simulink model "NGW_model"  (R2023b)
settings: Solver=ode4  StartTime=0  StopTime=0.5  FixedStep=1e-6  MaxStep=2e-4  RelTol=1e-7  AbsTol=1e-9
InitFcn:
  | NGW_init
values from neighbouring files (symbols this model uses):
  cL = 0    [NGW_init.m]    (also in NGW_test.m = 0.5)
  Flux = 0.01337    [NGW_init.m]
  i_ratio = p_m.i_ratio    [NGW_init.m]
  J_load = 4.53e-4    (= 0.000453)    [NGW_init.m]
  J_rotor = 1.0521e-4    (= 0.00010521)    [NGW_init.m]
  Kic = wc_i*1.05    (= 3298.67228627)    [NGW_init.m]
  Kis = Kps/Ti_s    [NGW_init.m]
  Kpc = wc_i*1.46e-3    (= 4.58672527424)    [NGW_init.m]
  Kps = wc_s*J_eq/Kt    [NGW_init.m]
  NtoW = 2*pi/60    (= 0.10471975512)    [NGW_init.m]
  P_n = 14    [NGW_init.m]
  TL_amp = 6    [NGW_init.m]
  TL_t0 = 0.2    [NGW_init.m]
  w_ref = 500    [NGW_init.m]
undefined symbols (not defined in the file or in its folder): NGW_params
libraries: slpidlib x6, spsDCVoltageSourceLib x2, spsUniversalBridgeLib x2, spsPermanentMagnetSynchronousMachineLib x2, spsSVPWMGenerator2LevelLib x2, sps_lib x1
settings Model: Creator=Administrator  LastModifiedBy=Administrator

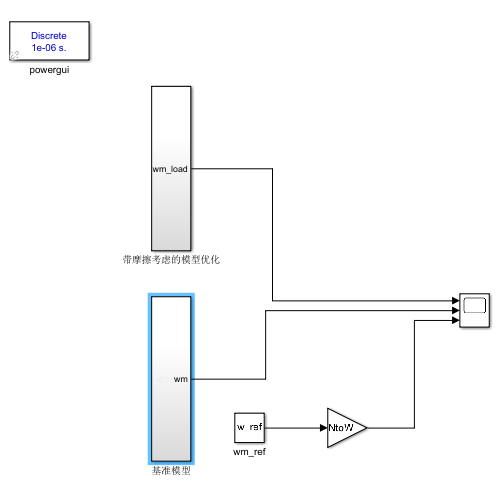
[thumbnail: Simulink's stored preview of the top-level diagram]
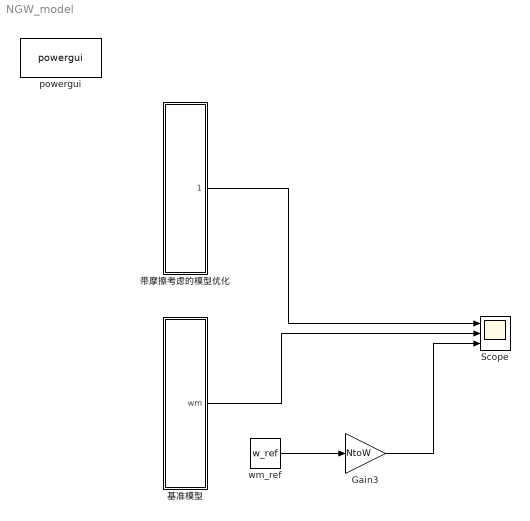
== system NGW_model ==
  Gain3 : Gain  Gain=NtoW
  Scope : Scope  NumInputPorts=3
  powergui : sps_lib/powergui  Priority=1  SimulationMode=Discrete  SampleTime=1e-6  frequency=60  Iterations=50  frequencyindice=0  Pbase=100e6  ErrMax=1e-4  UnitsV=kV  UnitsW=MW  buscounter=0  FunctionMessages=off  echomessages=off  EnableUseOfTLC=off  CurrentSourceSwitches=off  DisableSnubberDevices=off  DisableRonSwitches=off  DisableVfSwitches=off  DisplayEquations=off  AutomaticDiscreteSolvers=off  SolverType=Tustin/Backward Euler (TBE)  Interpol=off  ExternalGateDelay=off  methode=off  Ts=100  x0status=blocks  SPID=on  SwTol=0  HookPort=off  NonlinearTolerance=1e-4  nMaxIteration=100  ContinueOnMaxIteration=off  RestoreLinks=warning  ResistiveCurrentMeasurement=off  Frange=[0:2:500]  Ylog=off  Xlog=on  ShowGrid=off  save=off  variable=ZData  structure=0  ZoomFFT=off  StartTime=0.0  cycles=1  DisplayStyle=1  fundamental=60  FreqAxis=off  MaxFrequency=1000  frequencyindicesteady=1  RmsSteady=1  display=off
  wm_ref : Constant  Value=w_ref  SampleTime=-1
  基准模型 : Subsystem
  带摩擦考虑的模型优化 : Subsystem
  wires:
  带摩擦考虑的模型优化/1(wm_load) -> Scope/1
  基准模型/1(wm) -> Scope/2
  Gain3/1 -> Scope/3
  wm_ref/1 -> Gain3/1

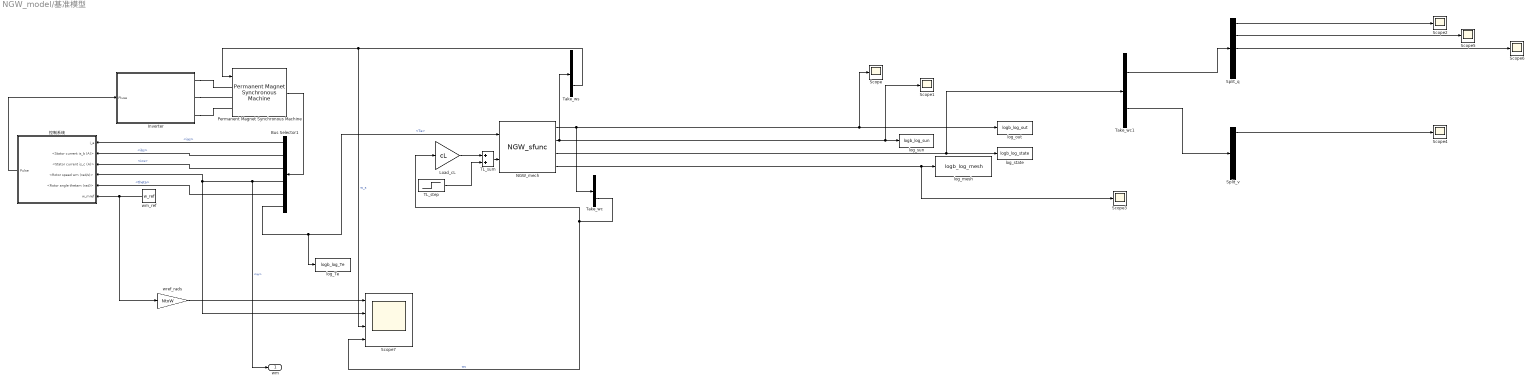
== system NGW_model/基准模型 ==
  Bus Selector1 : BusSelector  OutputSignals=ias,ibs,ics,w,theta,Te
  Inverter : Subsystem
  Load_cL : Gain  Gain=cL
  NGW_mech : M-S-Function  FunctionName=NGW_sfunc  Parameters=NGW_params(J_rotor, J_load)
  Permanent Magnet Synchronous Machine : spsPermanentMagnetSynchronousMachineLib/Permanent Magnet Synchronous Machine  NbPhases=3  FluxDistribution=Sinusoidal  RotorType=Round  MechanicalLoad=Speed w  PresetModel=No  ShowDetailedParameters=on  MeasurementBus=on  Resistance=1.05  Inductance=1.46e-3  dqInductances=[1.46e-3,1.46e-3]  La=0.000395  MachineConstant=Flux linkage established by magnets (V.s)  Flux=0.01337  VoltageCst=33.9507  TorqueCst=0.28077  Flat=120  Mechanical=[1.0521e-4 0 14 0]  PolePairs=14  InitialConditions=[0,0, 0,0]  InitialConditions5ph=[0 0 0 0 0 0]  RefAngle=Aligned with phase A axis (original Park)  IterativeDiscreteModel=Trapezoidal non iterative  TsBlock=-1  TsPowergui=0
  Scope{,1..6} (7 alike) : Scope
  Scope7 : Scope  NumInputPorts=4
  Split_q : Demux  Outputs=5
  Split_v : Demux  Outputs=5
  TL_step : Step  Time=TL_t0  After=TL_amp  SampleTime=0
  TL_sum : Sum
  Take_wc : Demux  Outputs=2
  Take_wc1 : Demux  Outputs=2
  Take_ws : Demux  Outputs=2
  log_Te : ToWorkspace  VariableName=logb_log_Te  SaveFormat=Timeseries  SampleTime=-1
  log_mesh : ToWorkspace  VariableName=logb_log_mesh  SaveFormat=Structure With Time  SampleTime=-1
  log_out : ToWorkspace  VariableName=logb_log_out  SaveFormat=Structure With Time  SampleTime=-1
  log_state : ToWorkspace  VariableName=logb_log_state  SaveFormat=Structure With Time  SampleTime=-1
  log_sun : ToWorkspace  VariableName=logb_log_sun  SaveFormat=Structure With Time  SampleTime=-1
  wm_ref : Constant  Value=w_ref  SampleTime=-1
  wref_rads : Gain  Gain=NtoW
  控制系统 : Subsystem
  wm : Outport
  wires:
  Split_v/1 -> Scope4/1
  Bus Selector1/5 -> 控制系统/5(<Rotor angle thetam (rad)>)  "<theta>"
  Split_q/2 -> Scope5/1
  Take_wc1/1 -> Split_q/1
  Bus Selector1/6 -> NGW_mech/1, log_Te/1  "<Te>"
  NGW_mech/1 -> log_out/1, Scope/1, Take_wc/1
  wm_ref/1 -> wref_rads/1, 控制系统/6(w_mref)
  Take_wc/2 -> Scope7/4, Load_cL/1  "wc"
  控制系统/1(Pulse) -> Inverter/1(Pluse)
  Take_wc1/2 -> Split_v/1
  Take_ws/2 -> Scope7/3, Permanent Magnet Synchronous Machine/1  "w_s"
  Split_q/1 -> Scope2/1
  Bus Selector1/1 -> 控制系统/1(i_a)  "<ias>"
  Split_q/3 -> Scope6/1
  NGW_mech/4 -> Scope3/1, log_mesh/1
  wref_rads/1 -> Scope7/1
  NGW_mech/2 -> Take_ws/1, Scope1/1, log_sun/1
  Bus Selector1/3 -> 控制系统/3(<Stator current is_c (A)>)  "<ics>"
  Bus Selector1/4 -> wm/1, Scope7/2, 控制系统/4(<Rotor speed wm (rad/s)>)  "<w>"
  NGW_mech/3 -> Take_wc1/1, log_state/1
  Permanent Magnet Synchronous Machine/1 -> Bus Selector1/1
  Bus Selector1/2 -> 控制系统/2(<Stator current is_b (A)>)  "<ibs>"
  Load_cL/1 -> TL_sum/1
  TL_step/1 -> TL_sum/2
  TL_sum/1 -> NGW_mech/2
  connections:
  Inverter/RConn2 -- Permanent Magnet Synchronous Machine/LConn2
  Inverter/RConn3 -- Permanent Magnet Synchronous Machine/LConn3
  Inverter/RConn1 -- Permanent Magnet Synchronous Machine/LConn1

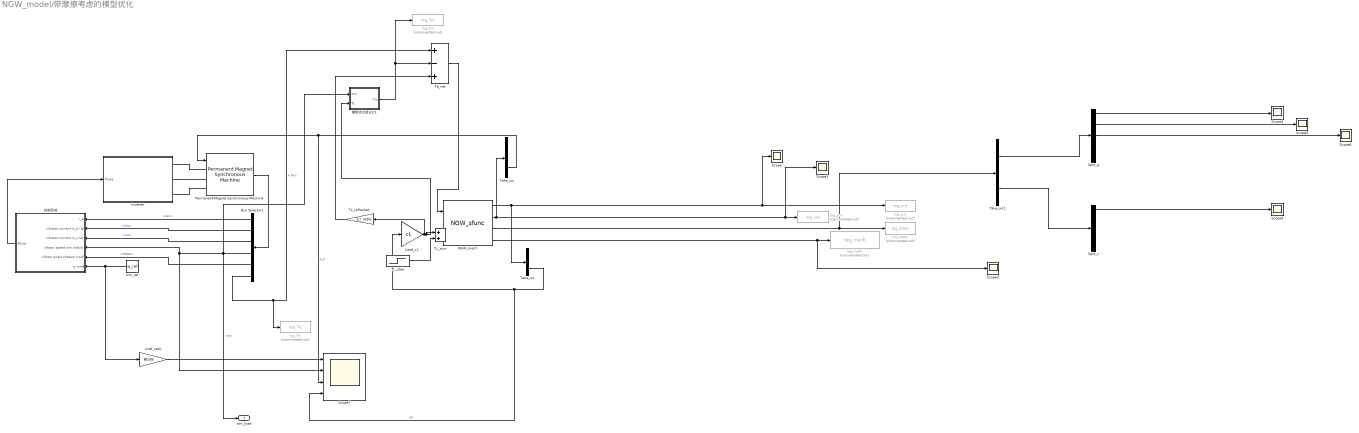
== system NGW_model/带摩擦考虑的模型优化 ==
  Bus Selector1 : BusSelector  OutputSignals=ias,ibs,ics,w,theta,Te
  Inverter : Subsystem
  Load_cL : Gain  Gain=cL
  NGW_mech : M-S-Function  FunctionName=NGW_sfunc  Parameters=NGW_params(J_rotor, J_load)
  Permanent Magnet Synchronous Machine : spsPermanentMagnetSynchronousMachineLib/Permanent Magnet Synchronous Machine  NbPhases=3  FluxDistribution=Sinusoidal  RotorType=Round  MechanicalLoad=Speed w  PresetModel=No  ShowDetailedParameters=on  MeasurementBus=on  Resistance=1.05  Inductance=1.46e-3  dqInductances=[1.46e-3,1.46e-3]  La=0.000395  MachineConstant=Flux linkage established by magnets (V.s)  Flux=0.01337  VoltageCst=33.9507  TorqueCst=0.28077  Flat=120  Mechanical=[1.0521e-4 0 14 0]  PolePairs=14  InitialConditions=[0,0, 0,0]  InitialConditions5ph=[0 0 0 0 0 0]  RefAngle=Aligned with phase A axis (original Park)  IterativeDiscreteModel=Trapezoidal non iterative  TsBlock=-1  TsPowergui=0
  Scope{,1..6} (7 alike) : Scope
  Scope7 : Scope  NumInputPorts=4
  Split_q : Demux  Outputs=5
  Split_v : Demux  Outputs=5
  TL_reflected : Gain  Gain=1/i_ratio
  TL_step : Step  Time=TL_t0  After=TL_amp  SampleTime=0
  TL_sum : Sum
  Take_wc : Demux  Outputs=2
  Take_wc1 : Demux  Outputs=2
  Take_ws : Demux  Outputs=2
  Te_net : Sum  Inputs=+-+
  log_Te : ToWorkspace  Commented=on  VariableName=log_Te  SaveFormat=Timeseries  SampleTime=-1
  log_Tm : ToWorkspace  Commented=on  VariableName=log_Tm  SaveFormat=Timeseries  SampleTime=-1
  log_mesh : ToWorkspace  Commented=on  VariableName=log_mesh  SaveFormat=Structure With Time  SampleTime=-1
  log_out : ToWorkspace  Commented=on  VariableName=log_out  SaveFormat=Structure With Time  SampleTime=-1
  log_state : ToWorkspace  Commented=on  VariableName=log_state  SaveFormat=Structure With Time  SampleTime=-1
  log_sun : ToWorkspace  Commented=on  VariableName=log_sun  SaveFormat=Structure With Time  SampleTime=-1
  wm_ref : Constant  Value=w_ref  SampleTime=-1
  wref_rads : Gain  Gain=NtoW
  控制系统 : Subsystem
  模型优化部分1/1 : Subsystem
  wm_load : Outport
  wires:
  Split_v/1 -> Scope4/1
  Bus Selector1/5 -> 控制系统/5(<Rotor angle thetam (rad)>)  "<theta>"
  Split_q/2 -> Scope5/1
  Take_wc1/1 -> Split_q/1
  Bus Selector1/6 -> log_Te/1, Te_net/1  "<Te>"
  模型优化部分1/1/1(Tm) -> log_Tm/1, Te_net/2
  NGW_mech/1 -> log_out/1, Scope/1, Take_wc/1
  wm_ref/1 -> wref_rads/1, 控制系统/6(w_mref)
  Take_wc/2 -> Scope7/4, Load_cL/1  "wc"
  Load_cL/1 -> 模型优化部分1/1/2(TL), TL_sum/1, TL_reflected/1
  控制系统/1(Pulse) -> Inverter/1(Pluse)
  Take_wc1/2 -> Split_v/1
  Take_ws/2 -> Scope7/3, Permanent Magnet Synchronous Machine/1  "w_s"
  TL_reflected/1 -> Te_net/3
  Split_q/1 -> Scope2/1
  Bus Selector1/1 -> 控制系统/1(i_a)  "<ias>"
  Split_q/3 -> Scope6/1
  NGW_mech/4 -> Scope3/1, log_mesh/1
  wref_rads/1 -> Scope7/1
  NGW_mech/2 -> Take_ws/1, Scope1/1, log_sun/1
  Bus Selector1/3 -> 控制系统/3(<Stator current is_c (A)>)  "<ics>"
  Bus Selector1/4 -> wm_load/1, 模型优化部分1/1/1(wm), Scope7/2, 控制系统/4(<Rotor speed wm (rad/s)>)  "<w>"
  NGW_mech/3 -> Take_wc1/1, log_state/1
  Te_net/1 -> NGW_mech/1
  Permanent Magnet Synchronous Machine/1 -> Bus Selector1/1
  Bus Selector1/2 -> 控制系统/2(<Stator current is_b (A)>)  "<ibs>"
  TL_step/1 -> TL_sum/2
  TL_sum/1 -> NGW_mech/2
  connections:
  Inverter/RConn2 -- Permanent Magnet Synchronous Machine/LConn2
  Inverter/RConn3 -- Permanent Magnet Synchronous Machine/LConn3
  Inverter/RConn1 -- Permanent Magnet Synchronous Machine/LConn1

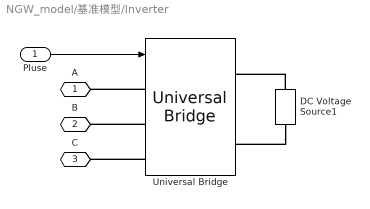
== system NGW_model/基准模型/Inverter ==
  Pluse : Inport
  DC Voltage Source1 : spsDCVoltageSourceLib/DC Voltage Source  Amplitude=72  Measurements=None
  Universal Bridge : spsUniversalBridgeLib/Universal Bridge  Arms=3  SnubberResistance=1e5  SnubberCapacitance=inf  Device=IGBT / Diodes  Ron=1e-3  Lon=0  ForwardVoltages="[  0  0  ]"  ForwardVoltage=0  GTOparameters=[ 10e-6 , 20e-6 ]  IGBTparameters=[ 1e-6 , 2e-6 ]  Measurements=None  Measurements_2=None  converterType=Rectifier
  A : PMIOPort  Side=Right
  B : PMIOPort  Port=2  Side=Right
  C : PMIOPort  Port=3  Side=Right
  wires:
  Pluse/1 -> Universal Bridge/1
  connections:
  Universal Bridge/LConn2 -- B/RConn1
  DC Voltage Source1/RConn1 -- Universal Bridge/RConn1
  DC Voltage Source1/LConn1 -- Universal Bridge/RConn2
  Universal Bridge/LConn3 -- C/RConn1
  Universal Bridge/LConn1 -- A/RConn1

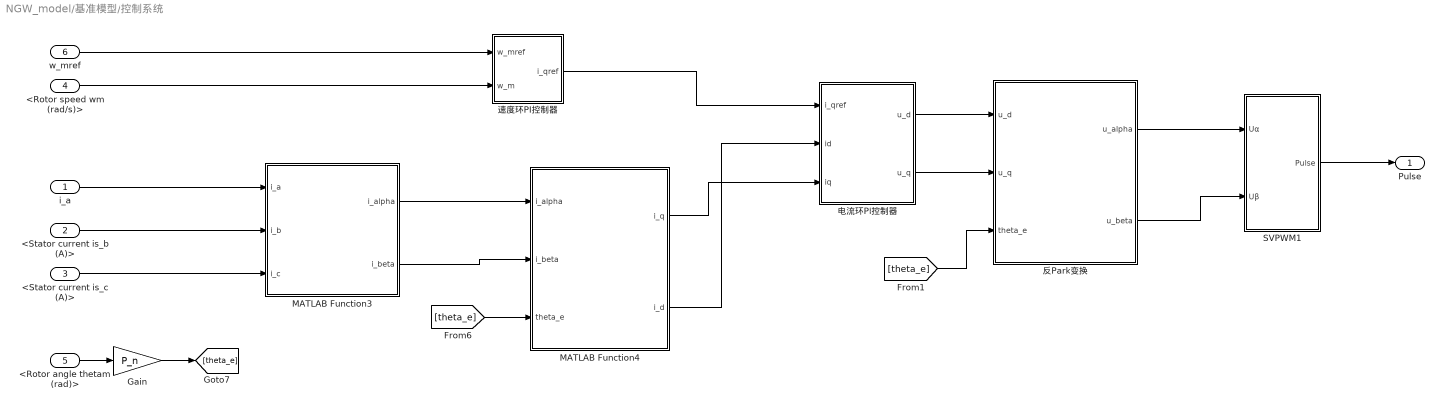
== system NGW_model/基准模型/控制系统 ==
  i_a : Inport
  <Stator current is_b (A)> : Inport  Port=2
  <Stator current is_c (A)> : Inport  Port=3
  <Rotor speed wm (rad/s)> : Inport  Port=4
  <Rotor angle thetam (rad)> : Inport  Port=5
  w_mref : Inport  Port=6
  Gain : Gain  Gain=P_n
  MATLAB Function3 : MATLAB Function  TreatAsAtomicUnit=on
  MATLAB Function4 : MATLAB Function  TreatAsAtomicUnit=on
  SVPWM1 : Subsystem
  反Park变换 : MATLAB Function  TreatAsAtomicUnit=on
  电流环PI控制器 : Subsystem
  速度环PI控制器 : Subsystem
  Pulse : Outport
  wires:
  i_a/1 -> MATLAB Function3/1(i_a)
  <Stator current is_b (A)>/1 -> MATLAB Function3/2(i_b)
  <Stator current is_c (A)>/1 -> MATLAB Function3/3(i_c)
  MATLAB Function3/1(i_alpha) -> MATLAB Function4/1(i_alpha)
  MATLAB Function3/2(i_beta) -> MATLAB Function4/2(i_beta)
  <Rotor angle thetam (rad)>/1 -> Gain/1
  Gain/1 -> [theta_e]
  [theta_e] -> MATLAB Function4/3(theta_e)
  MATLAB Function4/2(i_d) -> 电流环PI控制器/2(id)
  MATLAB Function4/1(i_q) -> 电流环PI控制器/3(iq)
  电流环PI控制器/1(u_d) -> 反Park变换/1(u_d)
  电流环PI控制器/2(u_q) -> 反Park变换/2(u_q)
  [theta_e] -> 反Park变换/3(theta_e)
  反Park变换/2(u_beta) -> SVPWM1/2(Uβ)
  反Park变换/1(u_alpha) -> SVPWM1/1(Uα)
  SVPWM1/1(Pulse) -> Pulse/1
  <Rotor speed wm (rad/s)>/1 -> 速度环PI控制器/2(w_m)
  速度环PI控制器/1(i_qref) -> 电流环PI控制器/1(i_qref)
  w_mref/1 -> 速度环PI控制器/1(w_mref)

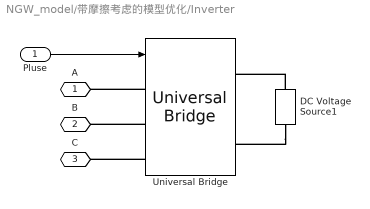
== system NGW_model/带摩擦考虑的模型优化/Inverter ==
  Pluse : Inport
  DC Voltage Source1 : spsDCVoltageSourceLib/DC Voltage Source  Amplitude=72  Measurements=None
  Universal Bridge : spsUniversalBridgeLib/Universal Bridge  Arms=3  SnubberResistance=1e5  SnubberCapacitance=inf  Device=IGBT / Diodes  Ron=1e-3  Lon=0  ForwardVoltages="[  0  0  ]"  ForwardVoltage=0  GTOparameters=[ 10e-6 , 20e-6 ]  IGBTparameters=[ 1e-6 , 2e-6 ]  Measurements=None  Measurements_2=None  converterType=Rectifier
  A : PMIOPort  Side=Right
  B : PMIOPort  Port=2  Side=Right
  C : PMIOPort  Port=3  Side=Right
  wires:
  Pluse/1 -> Universal Bridge/1
  connections:
  Universal Bridge/LConn2 -- B/RConn1
  DC Voltage Source1/RConn1 -- Universal Bridge/RConn1
  DC Voltage Source1/LConn1 -- Universal Bridge/RConn2
  Universal Bridge/LConn3 -- C/RConn1
  Universal Bridge/LConn1 -- A/RConn1

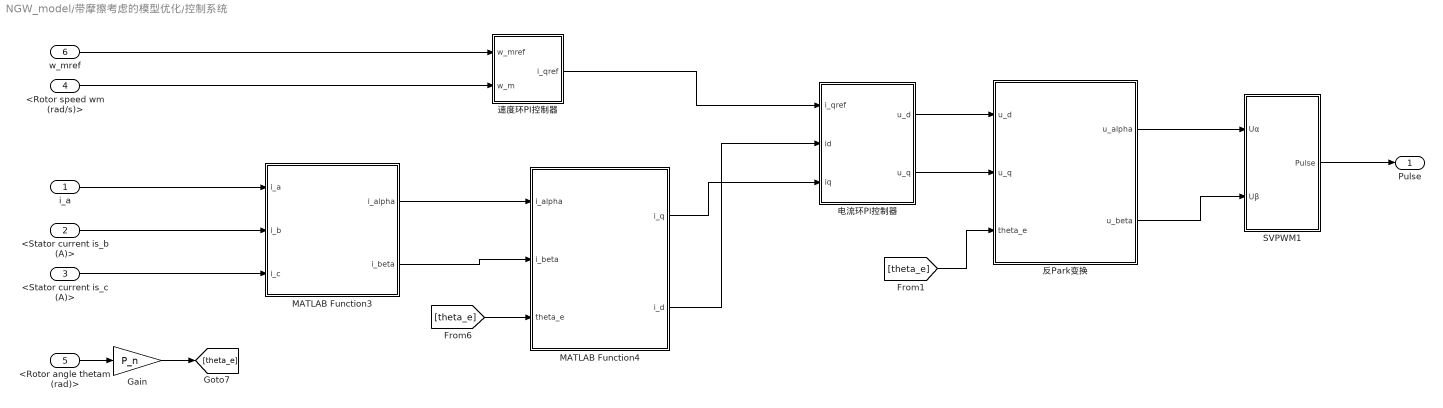
== system NGW_model/带摩擦考虑的模型优化/控制系统 ==
  i_a : Inport
  <Stator current is_b (A)> : Inport  Port=2
  <Stator current is_c (A)> : Inport  Port=3
  <Rotor speed wm (rad/s)> : Inport  Port=4
  <Rotor angle thetam (rad)> : Inport  Port=5
  w_mref : Inport  Port=6
  Gain : Gain  Gain=P_n
  MATLAB Function3 : MATLAB Function  TreatAsAtomicUnit=on
  MATLAB Function4 : MATLAB Function  TreatAsAtomicUnit=on
  SVPWM1 : Subsystem
  反Park变换 : MATLAB Function  TreatAsAtomicUnit=on
  电流环PI控制器 : Subsystem
  速度环PI控制器 : Subsystem
  Pulse : Outport
  wires:
  i_a/1 -> MATLAB Function3/1(i_a)
  <Stator current is_b (A)>/1 -> MATLAB Function3/2(i_b)
  <Stator current is_c (A)>/1 -> MATLAB Function3/3(i_c)
  MATLAB Function3/1(i_alpha) -> MATLAB Function4/1(i_alpha)
  MATLAB Function3/2(i_beta) -> MATLAB Function4/2(i_beta)
  <Rotor angle thetam (rad)>/1 -> Gain/1
  Gain/1 -> [theta_e]
  [theta_e] -> MATLAB Function4/3(theta_e)
  MATLAB Function4/2(i_d) -> 电流环PI控制器/2(id)
  MATLAB Function4/1(i_q) -> 电流环PI控制器/3(iq)
  电流环PI控制器/1(u_d) -> 反Park变换/1(u_d)
  电流环PI控制器/2(u_q) -> 反Park变换/2(u_q)
  [theta_e] -> 反Park变换/3(theta_e)
  反Park变换/2(u_beta) -> SVPWM1/2(Uβ)
  反Park变换/1(u_alpha) -> SVPWM1/1(Uα)
  SVPWM1/1(Pulse) -> Pulse/1
  <Rotor speed wm (rad/s)>/1 -> 速度环PI控制器/2(w_m)
  速度环PI控制器/1(i_qref) -> 电流环PI控制器/1(i_qref)
  w_mref/1 -> 速度环PI控制器/1(w_mref)

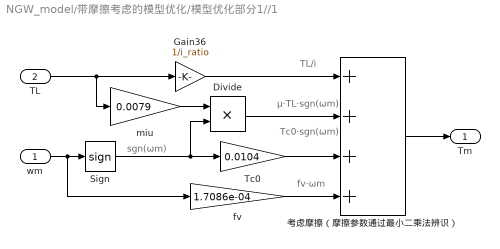
== system NGW_model/带摩擦考虑的模型优化/模型优化部分1//1 ==
  note: sgn(ωm)
  note: μ·TL·sgn(ωm)
  note: Tc0·sgn(ωm)
  note: fv·ωm
  note: TL/i
  wm : Inport
  TL : Inport  Port=2
  Divide : Product  Inputs=**
  Gain36 : Gain  Gain=1/i_ratio
  Sign : Signum
  Tc0 : Gain  Gain=0.0104
  fv : Gain  Gain=1.7086e-04
  miu : Gain  Gain=0.0079
  考虑摩擦（摩擦参数通过最小二乘法辨识） : Sum  Inputs=++++
  Tm : Outport
  wires:
  Gain36/1 -> 考虑摩擦（摩擦参数通过最小二乘法辨识）/1
  考虑摩擦（摩擦参数通过最小二乘法辨识）/1 -> Tm/1
  Tc0/1 -> 考虑摩擦（摩擦参数通过最小二乘法辨识）/3
  miu/1 -> Divide/1
  Sign/1 -> Divide/2, Tc0/1
  TL/1 -> miu/1, Gain36/1
  Divide/1 -> 考虑摩擦（摩擦参数通过最小二乘法辨识）/2
  fv/1 -> 考虑摩擦（摩擦参数通过最小二乘法辨识）/4
  wm/1 -> fv/1, Sign/1

== system NGW_model/基准模型/控制系统/SVPWM1 ==
  Uα : Inport
  Uβ : Inport  Port=2
  SVPWM Generator (2-Level) : spsSVPWMGenerator2LevelLib/SVPWM Generator (2-Level)  InputType=alpha-beta components  SwitchingPattern=Pattern #1  Fc=10000  ParUref=[0.8 -30 50]  Ts=1e-6
  Pulse : Outport
  wires:
  Uβ/1 -> SVPWM Generator (2-Level)/2
  Uα/1 -> SVPWM Generator (2-Level)/1
  SVPWM Generator (2-Level)/1 -> Pulse/1

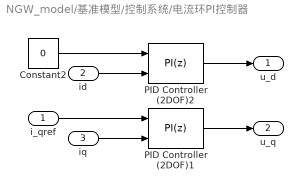
== system NGW_model/基准模型/控制系统/电流环PI控制器 ==
  i_qref : Inport
  id : Inport  Port=2
  iq : Inport  Port=3
  Constant2 : Constant  Value=0
  PID Controller (2DOF)1 : slpidlib/PID Controller (2DOF)  Controller=PI  Form=Parallel  TimeDomain=Discrete-time  UseExternalTs=off  SampleTime=5e-6  IntegratorMethod=Forward Euler  FilterMethod=Forward Euler  ControllerParametersSource=internal  P=Kpc  I=Kic  UseKiTs=off  D=0  N=100  UseFilter=on  b=1  c=1  TunerSelectOption=Transfer Function Based (PID Tuner App)  InitialConditionSource=internal  InitialConditionForIntegrator=0  InitialConditionForFilter=0  DifferentiatorICPrevScaledInput=0  ExternalReset=none  TrackingMode=off  Kt=1  LimitOutput=on  SatLimitsSource=internal  UpperSaturationLimit=72/sqrt(3)  LowerSaturationLimit=-72/sqrt(3)  LinearizeAsGain=on  AntiWindupMode=none  Kb=1  LimitIntegrator=off  UpperIntegratorSaturationLimit=inf  LowerIntegratorSaturationLimit=-inf  POutMin=[]  POutMax=[]  IOutMin=[]  IOutMax=[]  DOutMin=[]  DOutMax=[]  NOutMin=[]  NOutMax=[]  bOutMin=[]  bOutMax=[]  cOutMin=[]  cOutMax=[]  SumOutMin=[]  SumOutMax=[]  SaturationOutMin=[]  SaturationOutMax=[]  PParamMin=[]  PParamMax=[]  IParamMin=[]  IParamMax=[]  DParamMin=[]  DParamMax=[]  NParamMin=[]  NParamMax=[]  bParamMin=[]  bParamMax=[]  cParamMin=[]  cParamMax=[]  KbParamMin=[]  KbParamMax=[]  KtParamMin=[]  KtParamMax=[]  KbOutMin=[]  KbOutMax=[]  KtOutMin=[]  KtOutMax=[]  IntegratorOutMin=[]  IntegratorOutMax=[]  FilterOutMin=[]  FilterOutMax=[]  SumI1OutMin=[]  SumI1OutMax=[]  SumI2OutMin=[]  SumI2OutMax=[]  SumI3OutMin=[]  SumI3OutMax=[]  SumI4OutMin=[]  SumI4OutMax=[]  SumDOutMin=[]  SumDOutMax=[]  Sum1OutMin=[]  Sum1OutMax=[]  Sum2OutMin=[]  Sum2OutMax=[]  Sum3OutMin=[]  Sum3OutMax=[]  DifferentiatorOutMin=[]  DifferentiatorOutMax=[]  FilterDiffOutCoefMin=[]  FilterDiffOutCoefMax=[]  ReciprocalOutMin=[]  ReciprocalOutMax=[]  SumDenOutMin=[]  SumDenOutMax=[]  SumNumOutMin=[]  SumNumOutMax=[]  DivideOutMin=[]  DivideOutMax=[]  UdiffTsProdOutMin=[]  UdiffTsProdOutMax=[]  NTsProdOutMin=[]  NTsProdOutMax=[]  UintegralTsProdOutMin=[]  UintegralTsProdOutMax=[]  UngainTsProdOutMin=[]  UngainTsProdOutMax=[]  ClampingZeroOutDataTypeStr=Inherit: Inherit via back propagation  ClampingZeroOutMin=[]  ClampingZeroOutMax=[]  FilterDenConstantOutDataTypeStr=Inherit: Inherit via back propagation  FilterDenConstantOutMin=[]  FilterDenConstantOutMax=[]  PCopyOutDataTypeStr=Inherit: Inherit via back propagation  PCopyOutMin=[]  PCopyOutMax=[]  NCopyOutDataTypeStr=Inherit: Inherit via back propagation  NCopyOutMin=[]  NCopyOutMax=[]  IntegratorContinuousStateAttributes=''  IntegratorStateMustResolveToSignalObject=off  IntegratorRTWStateStorageClass=Auto  FilterContinuousStateAttributes=''  FilterStateMustResolveToSignalObject=off  FilterRTWStateStorageClass=Auto  ParallelPVariant=InternalParameters  IdealPVariant=Disabled  IVariant=InternalParameters  DVariant=Disabled  bVariant=InternalParameters  cVariant=Disabled  IntegratorVariant=Discrete  SatVariant=Enabled  AWVariant=Passthrough  PCopyVariant=Disabled  TRVariant=Disabled  FdbkBlocksVariant=Forward  IdealPFdbkVariant=Disabled  SatFdbkVariant=Disabled  DerivativeFilterVariant=Disabled  NVariant=Disabled  NCopyVariant=Disabled_SignalSpec  FilterICVariant=Disabled  IntegratorICVariant=InternalICs  ExternalResetVariant=Disabled  TRSumVariant=Passthrough  SumFdbkVariant=Disabled  SumVariant=Sum_PI  TsampFilterVariant=InternalTs  TsampNgainVariant=Passthrough  TsampIntegralVariant=Disabled_SignalSpec  ExternalSaturationOutDataTypeStr=Inherit: Same as second input
  PID Controller (2DOF)2 : slpidlib/PID Controller (2DOF)  Controller=PI  Form=Parallel  TimeDomain=Discrete-time  UseExternalTs=off  SampleTime=5e-6  IntegratorMethod=Forward Euler  FilterMethod=Forward Euler  ControllerParametersSource=internal  P=Kpc  I=Kic  UseKiTs=off  D=0  N=100  UseFilter=on  b=1  c=1  TunerSelectOption=Transfer Function Based (PID Tuner App)  InitialConditionSource=internal  InitialConditionForIntegrator=0  InitialConditionForFilter=0  DifferentiatorICPrevScaledInput=0  ExternalReset=none  TrackingMode=off  Kt=1  LimitOutput=on  SatLimitsSource=internal  UpperSaturationLimit=72/sqrt(3)  LowerSaturationLimit=-72/sqrt(3)  LinearizeAsGain=on  AntiWindupMode=none  Kb=1  LimitIntegrator=off  UpperIntegratorSaturationLimit=inf  LowerIntegratorSaturationLimit=-inf  POutMin=[]  POutMax=[]  IOutMin=[]  IOutMax=[]  DOutMin=[]  DOutMax=[]  NOutMin=[]  NOutMax=[]  bOutMin=[]  bOutMax=[]  cOutMin=[]  cOutMax=[]  SumOutMin=[]  SumOutMax=[]  SaturationOutMin=[]  SaturationOutMax=[]  PParamMin=[]  PParamMax=[]  IParamMin=[]  IParamMax=[]  DParamMin=[]  DParamMax=[]  NParamMin=[]  NParamMax=[]  bParamMin=[]  bParamMax=[]  cParamMin=[]  cParamMax=[]  KbParamMin=[]  KbParamMax=[]  KtParamMin=[]  KtParamMax=[]  KbOutMin=[]  KbOutMax=[]  KtOutMin=[]  KtOutMax=[]  IntegratorOutMin=[]  IntegratorOutMax=[]  FilterOutMin=[]  FilterOutMax=[]  SumI1OutMin=[]  SumI1OutMax=[]  SumI2OutMin=[]  SumI2OutMax=[]  SumI3OutMin=[]  SumI3OutMax=[]  SumI4OutMin=[]  SumI4OutMax=[]  SumDOutMin=[]  SumDOutMax=[]  Sum1OutMin=[]  Sum1OutMax=[]  Sum2OutMin=[]  Sum2OutMax=[]  Sum3OutMin=[]  Sum3OutMax=[]  DifferentiatorOutMin=[]  DifferentiatorOutMax=[]  FilterDiffOutCoefMin=[]  FilterDiffOutCoefMax=[]  ReciprocalOutMin=[]  ReciprocalOutMax=[]  SumDenOutMin=[]  SumDenOutMax=[]  SumNumOutMin=[]  SumNumOutMax=[]  DivideOutMin=[]  DivideOutMax=[]  UdiffTsProdOutMin=[]  UdiffTsProdOutMax=[]  NTsProdOutMin=[]  NTsProdOutMax=[]  UintegralTsProdOutMin=[]  UintegralTsProdOutMax=[]  UngainTsProdOutMin=[]  UngainTsProdOutMax=[]  ClampingZeroOutDataTypeStr=Inherit: Inherit via back propagation  ClampingZeroOutMin=[]  ClampingZeroOutMax=[]  FilterDenConstantOutDataTypeStr=Inherit: Inherit via back propagation  FilterDenConstantOutMin=[]  FilterDenConstantOutMax=[]  PCopyOutDataTypeStr=Inherit: Inherit via back propagation  PCopyOutMin=[]  PCopyOutMax=[]  NCopyOutDataTypeStr=Inherit: Inherit via back propagation  NCopyOutMin=[]  NCopyOutMax=[]  IntegratorContinuousStateAttributes=''  IntegratorStateMustResolveToSignalObject=off  IntegratorRTWStateStorageClass=Auto  FilterContinuousStateAttributes=''  FilterStateMustResolveToSignalObject=off  FilterRTWStateStorageClass=Auto  ParallelPVariant=InternalParameters  IdealPVariant=Disabled  IVariant=InternalParameters  DVariant=Disabled  bVariant=InternalParameters  cVariant=Disabled  IntegratorVariant=Discrete  SatVariant=Enabled  AWVariant=Passthrough  PCopyVariant=Disabled  TRVariant=Disabled  FdbkBlocksVariant=Forward  IdealPFdbkVariant=Disabled  SatFdbkVariant=Disabled  DerivativeFilterVariant=Disabled  NVariant=Disabled  NCopyVariant=Disabled_SignalSpec  FilterICVariant=Disabled  IntegratorICVariant=InternalICs  ExternalResetVariant=Disabled  TRSumVariant=Passthrough  SumFdbkVariant=Disabled  SumVariant=Sum_PI  TsampFilterVariant=InternalTs  TsampNgainVariant=Passthrough  TsampIntegralVariant=Disabled_SignalSpec  ExternalSaturationOutDataTypeStr=Inherit: Same as second input
  u_d : Outport
  u_q : Outport  Port=2
  wires:
  PID Controller (2DOF)1/1 -> u_q/1
  id/1 -> PID Controller (2DOF)2/2
  iq/1 -> PID Controller (2DOF)1/2
  Constant2/1 -> PID Controller (2DOF)2/1
  PID Controller (2DOF)2/1 -> u_d/1
  i_qref/1 -> PID Controller (2DOF)1/1

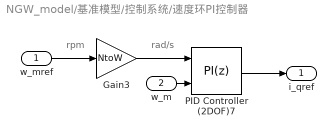
== system NGW_model/基准模型/控制系统/速度环PI控制器 ==
  note: rad/s
  note: rpm
  w_mref : Inport
  w_m : Inport  Port=2
  Gain3 : Gain  Gain=NtoW
  PID Controller (2DOF)7 : slpidlib/PID Controller (2DOF)  Controller=PI  Form=Parallel  TimeDomain=Discrete-time  UseExternalTs=off  SampleTime=5e-6  IntegratorMethod=Forward Euler  FilterMethod=Forward Euler  ControllerParametersSource=internal  P=Kps  I=Kis  UseKiTs=off  D=0  N=100  UseFilter=on  b=1  c=1  TunerSelectOption=Transfer Function Based (PID Tuner App)  InitialConditionSource=internal  InitialConditionForIntegrator=0  InitialConditionForFilter=0  DifferentiatorICPrevScaledInput=0  ExternalReset=none  TrackingMode=off  Kt=1  LimitOutput=on  SatLimitsSource=internal  UpperSaturationLimit=23  LowerSaturationLimit=-23  LinearizeAsGain=on  AntiWindupMode=none  Kb=1  LimitIntegrator=off  UpperIntegratorSaturationLimit=inf  LowerIntegratorSaturationLimit=-inf  POutMin=[]  POutMax=[]  IOutMin=[]  IOutMax=[]  DOutMin=[]  DOutMax=[]  NOutMin=[]  NOutMax=[]  bOutMin=[]  bOutMax=[]  cOutMin=[]  cOutMax=[]  SumOutMin=[]  SumOutMax=[]  SaturationOutMin=[]  SaturationOutMax=[]  PParamMin=[]  PParamMax=[]  IParamMin=[]  IParamMax=[]  DParamMin=[]  DParamMax=[]  NParamMin=[]  NParamMax=[]  bParamMin=[]  bParamMax=[]  cParamMin=[]  cParamMax=[]  KbParamMin=[]  KbParamMax=[]  KtParamMin=[]  KtParamMax=[]  KbOutMin=[]  KbOutMax=[]  KtOutMin=[]  KtOutMax=[]  IntegratorOutMin=[]  IntegratorOutMax=[]  FilterOutMin=[]  FilterOutMax=[]  SumI1OutMin=[]  SumI1OutMax=[]  SumI2OutMin=[]  SumI2OutMax=[]  SumI3OutMin=[]  SumI3OutMax=[]  SumI4OutMin=[]  SumI4OutMax=[]  SumDOutMin=[]  SumDOutMax=[]  Sum1OutMin=[]  Sum1OutMax=[]  Sum2OutMin=[]  Sum2OutMax=[]  Sum3OutMin=[]  Sum3OutMax=[]  DifferentiatorOutMin=[]  DifferentiatorOutMax=[]  FilterDiffOutCoefMin=[]  FilterDiffOutCoefMax=[]  ReciprocalOutMin=[]  ReciprocalOutMax=[]  SumDenOutMin=[]  SumDenOutMax=[]  SumNumOutMin=[]  SumNumOutMax=[]  DivideOutMin=[]  DivideOutMax=[]  UdiffTsProdOutMin=[]  UdiffTsProdOutMax=[]  NTsProdOutMin=[]  NTsProdOutMax=[]  UintegralTsProdOutMin=[]  UintegralTsProdOutMax=[]  UngainTsProdOutMin=[]  UngainTsProdOutMax=[]  ClampingZeroOutDataTypeStr=Inherit: Inherit via back propagation  ClampingZeroOutMin=[]  ClampingZeroOutMax=[]  FilterDenConstantOutDataTypeStr=Inherit: Inherit via back propagation  FilterDenConstantOutMin=[]  FilterDenConstantOutMax=[]  PCopyOutDataTypeStr=Inherit: Inherit via back propagation  PCopyOutMin=[]  PCopyOutMax=[]  NCopyOutDataTypeStr=Inherit: Inherit via back propagation  NCopyOutMin=[]  NCopyOutMax=[]  IntegratorContinuousStateAttributes=''  IntegratorStateMustResolveToSignalObject=off  IntegratorRTWStateStorageClass=Auto  FilterContinuousStateAttributes=''  FilterStateMustResolveToSignalObject=off  FilterRTWStateStorageClass=Auto  ParallelPVariant=InternalParameters  IdealPVariant=Disabled  IVariant=InternalParameters  DVariant=Disabled  bVariant=InternalParameters  cVariant=Disabled  IntegratorVariant=Discrete  SatVariant=Enabled  AWVariant=Passthrough  PCopyVariant=Disabled  TRVariant=Disabled  FdbkBlocksVariant=Forward  IdealPFdbkVariant=Disabled  SatFdbkVariant=Disabled  DerivativeFilterVariant=Disabled  NVariant=Disabled  NCopyVariant=Disabled_SignalSpec  FilterICVariant=Disabled  IntegratorICVariant=InternalICs  ExternalResetVariant=Disabled  TRSumVariant=Passthrough  SumFdbkVariant=Disabled  SumVariant=Sum_PI  TsampFilterVariant=InternalTs  TsampNgainVariant=Passthrough  TsampIntegralVariant=Disabled_SignalSpec  ExternalSaturationOutDataTypeStr=Inherit: Same as second input
  i_qref : Outport
  wires:
  Gain3/1 -> PID Controller (2DOF)7/1
  w_mref/1 -> Gain3/1
  PID Controller (2DOF)7/1 -> i_qref/1
  w_m/1 -> PID Controller (2DOF)7/2

== system NGW_model/带摩擦考虑的模型优化/控制系统/SVPWM1 ==
  Uα : Inport
  Uβ : Inport  Port=2
  SVPWM Generator (2-Level) : spsSVPWMGenerator2LevelLib/SVPWM Generator (2-Level)  InputType=alpha-beta components  SwitchingPattern=Pattern #1  Fc=10000  ParUref=[0.8 -30 50]  Ts=1e-6
  Pulse : Outport
  wires:
  Uβ/1 -> SVPWM Generator (2-Level)/2
  Uα/1 -> SVPWM Generator (2-Level)/1
  SVPWM Generator (2-Level)/1 -> Pulse/1

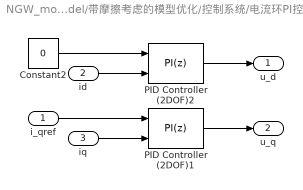
== system NGW_model/带摩擦考虑的模型优化/控制系统/电流环PI控制器 ==
  i_qref : Inport
  id : Inport  Port=2
  iq : Inport  Port=3
  Constant2 : Constant  Value=0
  PID Controller (2DOF)1 : slpidlib/PID Controller (2DOF)  Controller=PI  Form=Parallel  TimeDomain=Discrete-time  UseExternalTs=off  SampleTime=5e-6  IntegratorMethod=Forward Euler  FilterMethod=Forward Euler  ControllerParametersSource=internal  P=Kpc  I=Kic  UseKiTs=off  D=0  N=100  UseFilter=on  b=1  c=1  TunerSelectOption=Transfer Function Based (PID Tuner App)  InitialConditionSource=internal  InitialConditionForIntegrator=0  InitialConditionForFilter=0  DifferentiatorICPrevScaledInput=0  ExternalReset=none  TrackingMode=off  Kt=1  LimitOutput=on  SatLimitsSource=internal  UpperSaturationLimit=72/sqrt(3)  LowerSaturationLimit=-72/sqrt(3)  LinearizeAsGain=on  AntiWindupMode=none  Kb=1  LimitIntegrator=off  UpperIntegratorSaturationLimit=inf  LowerIntegratorSaturationLimit=-inf  POutMin=[]  POutMax=[]  IOutMin=[]  IOutMax=[]  DOutMin=[]  DOutMax=[]  NOutMin=[]  NOutMax=[]  bOutMin=[]  bOutMax=[]  cOutMin=[]  cOutMax=[]  SumOutMin=[]  SumOutMax=[]  SaturationOutMin=[]  SaturationOutMax=[]  PParamMin=[]  PParamMax=[]  IParamMin=[]  IParamMax=[]  DParamMin=[]  DParamMax=[]  NParamMin=[]  NParamMax=[]  bParamMin=[]  bParamMax=[]  cParamMin=[]  cParamMax=[]  KbParamMin=[]  KbParamMax=[]  KtParamMin=[]  KtParamMax=[]  KbOutMin=[]  KbOutMax=[]  KtOutMin=[]  KtOutMax=[]  IntegratorOutMin=[]  IntegratorOutMax=[]  FilterOutMin=[]  FilterOutMax=[]  SumI1OutMin=[]  SumI1OutMax=[]  SumI2OutMin=[]  SumI2OutMax=[]  SumI3OutMin=[]  SumI3OutMax=[]  SumI4OutMin=[]  SumI4OutMax=[]  SumDOutMin=[]  SumDOutMax=[]  Sum1OutMin=[]  Sum1OutMax=[]  Sum2OutMin=[]  Sum2OutMax=[]  Sum3OutMin=[]  Sum3OutMax=[]  DifferentiatorOutMin=[]  DifferentiatorOutMax=[]  FilterDiffOutCoefMin=[]  FilterDiffOutCoefMax=[]  ReciprocalOutMin=[]  ReciprocalOutMax=[]  SumDenOutMin=[]  SumDenOutMax=[]  SumNumOutMin=[]  SumNumOutMax=[]  DivideOutMin=[]  DivideOutMax=[]  UdiffTsProdOutMin=[]  UdiffTsProdOutMax=[]  NTsProdOutMin=[]  NTsProdOutMax=[]  UintegralTsProdOutMin=[]  UintegralTsProdOutMax=[]  UngainTsProdOutMin=[]  UngainTsProdOutMax=[]  ClampingZeroOutDataTypeStr=Inherit: Inherit via back propagation  ClampingZeroOutMin=[]  ClampingZeroOutMax=[]  FilterDenConstantOutDataTypeStr=Inherit: Inherit via back propagation  FilterDenConstantOutMin=[]  FilterDenConstantOutMax=[]  PCopyOutDataTypeStr=Inherit: Inherit via back propagation  PCopyOutMin=[]  PCopyOutMax=[]  NCopyOutDataTypeStr=Inherit: Inherit via back propagation  NCopyOutMin=[]  NCopyOutMax=[]  IntegratorContinuousStateAttributes=''  IntegratorStateMustResolveToSignalObject=off  IntegratorRTWStateStorageClass=Auto  FilterContinuousStateAttributes=''  FilterStateMustResolveToSignalObject=off  FilterRTWStateStorageClass=Auto  ParallelPVariant=InternalParameters  IdealPVariant=Disabled  IVariant=InternalParameters  DVariant=Disabled  bVariant=InternalParameters  cVariant=Disabled  IntegratorVariant=Discrete  SatVariant=Enabled  AWVariant=Passthrough  PCopyVariant=Disabled  TRVariant=Disabled  FdbkBlocksVariant=Forward  IdealPFdbkVariant=Disabled  SatFdbkVariant=Disabled  DerivativeFilterVariant=Disabled  NVariant=Disabled  NCopyVariant=Disabled_SignalSpec  FilterICVariant=Disabled  IntegratorICVariant=InternalICs  ExternalResetVariant=Disabled  TRSumVariant=Passthrough  SumFdbkVariant=Disabled  SumVariant=Sum_PI  TsampFilterVariant=InternalTs  TsampNgainVariant=Passthrough  TsampIntegralVariant=Disabled_SignalSpec  ExternalSaturationOutDataTypeStr=Inherit: Same as second input
  PID Controller (2DOF)2 : slpidlib/PID Controller (2DOF)  Controller=PI  Form=Parallel  TimeDomain=Discrete-time  UseExternalTs=off  SampleTime=5e-6  IntegratorMethod=Forward Euler  FilterMethod=Forward Euler  ControllerParametersSource=internal  P=Kpc  I=Kic  UseKiTs=off  D=0  N=100  UseFilter=on  b=1  c=1  TunerSelectOption=Transfer Function Based (PID Tuner App)  InitialConditionSource=internal  InitialConditionForIntegrator=0  InitialConditionForFilter=0  DifferentiatorICPrevScaledInput=0  ExternalReset=none  TrackingMode=off  Kt=1  LimitOutput=on  SatLimitsSource=internal  UpperSaturationLimit=72/sqrt(3)  LowerSaturationLimit=-72/sqrt(3)  LinearizeAsGain=on  AntiWindupMode=none  Kb=1  LimitIntegrator=off  UpperIntegratorSaturationLimit=inf  LowerIntegratorSaturationLimit=-inf  POutMin=[]  POutMax=[]  IOutMin=[]  IOutMax=[]  DOutMin=[]  DOutMax=[]  NOutMin=[]  NOutMax=[]  bOutMin=[]  bOutMax=[]  cOutMin=[]  cOutMax=[]  SumOutMin=[]  SumOutMax=[]  SaturationOutMin=[]  SaturationOutMax=[]  PParamMin=[]  PParamMax=[]  IParamMin=[]  IParamMax=[]  DParamMin=[]  DParamMax=[]  NParamMin=[]  NParamMax=[]  bParamMin=[]  bParamMax=[]  cParamMin=[]  cParamMax=[]  KbParamMin=[]  KbParamMax=[]  KtParamMin=[]  KtParamMax=[]  KbOutMin=[]  KbOutMax=[]  KtOutMin=[]  KtOutMax=[]  IntegratorOutMin=[]  IntegratorOutMax=[]  FilterOutMin=[]  FilterOutMax=[]  SumI1OutMin=[]  SumI1OutMax=[]  SumI2OutMin=[]  SumI2OutMax=[]  SumI3OutMin=[]  SumI3OutMax=[]  SumI4OutMin=[]  SumI4OutMax=[]  SumDOutMin=[]  SumDOutMax=[]  Sum1OutMin=[]  Sum1OutMax=[]  Sum2OutMin=[]  Sum2OutMax=[]  Sum3OutMin=[]  Sum3OutMax=[]  DifferentiatorOutMin=[]  DifferentiatorOutMax=[]  FilterDiffOutCoefMin=[]  FilterDiffOutCoefMax=[]  ReciprocalOutMin=[]  ReciprocalOutMax=[]  SumDenOutMin=[]  SumDenOutMax=[]  SumNumOutMin=[]  SumNumOutMax=[]  DivideOutMin=[]  DivideOutMax=[]  UdiffTsProdOutMin=[]  UdiffTsProdOutMax=[]  NTsProdOutMin=[]  NTsProdOutMax=[]  UintegralTsProdOutMin=[]  UintegralTsProdOutMax=[]  UngainTsProdOutMin=[]  UngainTsProdOutMax=[]  ClampingZeroOutDataTypeStr=Inherit: Inherit via back propagation  ClampingZeroOutMin=[]  ClampingZeroOutMax=[]  FilterDenConstantOutDataTypeStr=Inherit: Inherit via back propagation  FilterDenConstantOutMin=[]  FilterDenConstantOutMax=[]  PCopyOutDataTypeStr=Inherit: Inherit via back propagation  PCopyOutMin=[]  PCopyOutMax=[]  NCopyOutDataTypeStr=Inherit: Inherit via back propagation  NCopyOutMin=[]  NCopyOutMax=[]  IntegratorContinuousStateAttributes=''  IntegratorStateMustResolveToSignalObject=off  IntegratorRTWStateStorageClass=Auto  FilterContinuousStateAttributes=''  FilterStateMustResolveToSignalObject=off  FilterRTWStateStorageClass=Auto  ParallelPVariant=InternalParameters  IdealPVariant=Disabled  IVariant=InternalParameters  DVariant=Disabled  bVariant=InternalParameters  cVariant=Disabled  IntegratorVariant=Discrete  SatVariant=Enabled  AWVariant=Passthrough  PCopyVariant=Disabled  TRVariant=Disabled  FdbkBlocksVariant=Forward  IdealPFdbkVariant=Disabled  SatFdbkVariant=Disabled  DerivativeFilterVariant=Disabled  NVariant=Disabled  NCopyVariant=Disabled_SignalSpec  FilterICVariant=Disabled  IntegratorICVariant=InternalICs  ExternalResetVariant=Disabled  TRSumVariant=Passthrough  SumFdbkVariant=Disabled  SumVariant=Sum_PI  TsampFilterVariant=InternalTs  TsampNgainVariant=Passthrough  TsampIntegralVariant=Disabled_SignalSpec  ExternalSaturationOutDataTypeStr=Inherit: Same as second input
  u_d : Outport
  u_q : Outport  Port=2
  wires:
  PID Controller (2DOF)1/1 -> u_q/1
  id/1 -> PID Controller (2DOF)2/2
  iq/1 -> PID Controller (2DOF)1/2
  Constant2/1 -> PID Controller (2DOF)2/1
  PID Controller (2DOF)2/1 -> u_d/1
  i_qref/1 -> PID Controller (2DOF)1/1

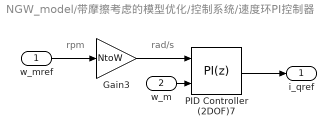
== system NGW_model/带摩擦考虑的模型优化/控制系统/速度环PI控制器 ==
  note: rad/s
  note: rpm
  w_mref : Inport
  w_m : Inport  Port=2
  Gain3 : Gain  Gain=NtoW
  PID Controller (2DOF)7 : slpidlib/PID Controller (2DOF)  Controller=PI  Form=Parallel  TimeDomain=Discrete-time  UseExternalTs=off  SampleTime=5e-6  IntegratorMethod=Forward Euler  FilterMethod=Forward Euler  ControllerParametersSource=internal  P=Kps  I=Kis  UseKiTs=off  D=0  N=100  UseFilter=on  b=1  c=1  TunerSelectOption=Transfer Function Based (PID Tuner App)  InitialConditionSource=internal  InitialConditionForIntegrator=0  InitialConditionForFilter=0  DifferentiatorICPrevScaledInput=0  ExternalReset=none  TrackingMode=off  Kt=1  LimitOutput=on  SatLimitsSource=internal  UpperSaturationLimit=23  LowerSaturationLimit=-23  LinearizeAsGain=on  AntiWindupMode=none  Kb=1  LimitIntegrator=off  UpperIntegratorSaturationLimit=inf  LowerIntegratorSaturationLimit=-inf  POutMin=[]  POutMax=[]  IOutMin=[]  IOutMax=[]  DOutMin=[]  DOutMax=[]  NOutMin=[]  NOutMax=[]  bOutMin=[]  bOutMax=[]  cOutMin=[]  cOutMax=[]  SumOutMin=[]  SumOutMax=[]  SaturationOutMin=[]  SaturationOutMax=[]  PParamMin=[]  PParamMax=[]  IParamMin=[]  IParamMax=[]  DParamMin=[]  DParamMax=[]  NParamMin=[]  NParamMax=[]  bParamMin=[]  bParamMax=[]  cParamMin=[]  cParamMax=[]  KbParamMin=[]  KbParamMax=[]  KtParamMin=[]  KtParamMax=[]  KbOutMin=[]  KbOutMax=[]  KtOutMin=[]  KtOutMax=[]  IntegratorOutMin=[]  IntegratorOutMax=[]  FilterOutMin=[]  FilterOutMax=[]  SumI1OutMin=[]  SumI1OutMax=[]  SumI2OutMin=[]  SumI2OutMax=[]  SumI3OutMin=[]  SumI3OutMax=[]  SumI4OutMin=[]  SumI4OutMax=[]  SumDOutMin=[]  SumDOutMax=[]  Sum1OutMin=[]  Sum1OutMax=[]  Sum2OutMin=[]  Sum2OutMax=[]  Sum3OutMin=[]  Sum3OutMax=[]  DifferentiatorOutMin=[]  DifferentiatorOutMax=[]  FilterDiffOutCoefMin=[]  FilterDiffOutCoefMax=[]  ReciprocalOutMin=[]  ReciprocalOutMax=[]  SumDenOutMin=[]  SumDenOutMax=[]  SumNumOutMin=[]  SumNumOutMax=[]  DivideOutMin=[]  DivideOutMax=[]  UdiffTsProdOutMin=[]  UdiffTsProdOutMax=[]  NTsProdOutMin=[]  NTsProdOutMax=[]  UintegralTsProdOutMin=[]  UintegralTsProdOutMax=[]  UngainTsProdOutMin=[]  UngainTsProdOutMax=[]  ClampingZeroOutDataTypeStr=Inherit: Inherit via back propagation  ClampingZeroOutMin=[]  ClampingZeroOutMax=[]  FilterDenConstantOutDataTypeStr=Inherit: Inherit via back propagation  FilterDenConstantOutMin=[]  FilterDenConstantOutMax=[]  PCopyOutDataTypeStr=Inherit: Inherit via back propagation  PCopyOutMin=[]  PCopyOutMax=[]  NCopyOutDataTypeStr=Inherit: Inherit via back propagation  NCopyOutMin=[]  NCopyOutMax=[]  IntegratorContinuousStateAttributes=''  IntegratorStateMustResolveToSignalObject=off  IntegratorRTWStateStorageClass=Auto  FilterContinuousStateAttributes=''  FilterStateMustResolveToSignalObject=off  FilterRTWStateStorageClass=Auto  ParallelPVariant=InternalParameters  IdealPVariant=Disabled  IVariant=InternalParameters  DVariant=Disabled  bVariant=InternalParameters  cVariant=Disabled  IntegratorVariant=Discrete  SatVariant=Enabled  AWVariant=Passthrough  PCopyVariant=Disabled  TRVariant=Disabled  FdbkBlocksVariant=Forward  IdealPFdbkVariant=Disabled  SatFdbkVariant=Disabled  DerivativeFilterVariant=Disabled  NVariant=Disabled  NCopyVariant=Disabled_SignalSpec  FilterICVariant=Disabled  IntegratorICVariant=InternalICs  ExternalResetVariant=Disabled  TRSumVariant=Passthrough  SumFdbkVariant=Disabled  SumVariant=Sum_PI  TsampFilterVariant=InternalTs  TsampNgainVariant=Passthrough  TsampIntegralVariant=Disabled_SignalSpec  ExternalSaturationOutDataTypeStr=Inherit: Same as second input
  i_qref : Outport
  wires:
  Gain3/1 -> PID Controller (2DOF)7/1
  w_mref/1 -> Gain3/1
  PID Controller (2DOF)7/1 -> i_qref/1
  w_m/1 -> PID Controller (2DOF)7/2

== matlab function NGW_model/基准模型/控制系统/MATLAB Function3 ==
  data: i_a input; i_alpha output; i_b input; i_c input; i_beta output
function [i_alpha, i_beta] = clarke(i_a,i_b,i_c)

i_alpha=(i_a-1/2*i_b-1/2*i_c)*2/3;
i_beta=(sqrt(3)/2*i_b-sqrt(3)/2*i_c)*2/3;

== matlab function NGW_model/基准模型/控制系统/MATLAB Function4 ==
  data: i_q output; i_alpha input; i_d output; i_beta input; theta_e input
function [i_q,i_d] = park(i_alpha,i_beta,theta_e)

i_d=i_alpha*cos(theta_e)+i_beta*sin(theta_e);
i_q=-i_alpha*sin(theta_e)+i_beta*cos(theta_e);
% I_d=-(I_alph.*cos(theta)+I_beta.*sin(theta));
% I_q= -(-I_alph.*sin(theta)+I_beta.*cos(theta));

== matlab function NGW_model/基准模型/控制系统/反Park变换 ==
  data: u_d input; u_q input; u_alpha output; u_beta output; theta_e input
function [u_alpha, u_beta]  = inv_park(u_d,u_q,theta_e)

u_alpha=cos(theta_e)*u_d-sin(theta_e)*u_q;
u_beta=sin(theta_e)*u_d+cos(theta_e)*u_q;

end

== matlab function NGW_model/带摩擦考虑的模型优化/控制系统/MATLAB Function3 ==
  data: i_a input; i_alpha output; i_b input; i_c input; i_beta output
function [i_alpha, i_beta] = clarke(i_a,i_b,i_c)

i_alpha=(i_a-1/2*i_b-1/2*i_c)*2/3;
i_beta=(sqrt(3)/2*i_b-sqrt(3)/2*i_c)*2/3;

== matlab function NGW_model/带摩擦考虑的模型优化/控制系统/MATLAB Function4 ==
  data: i_q output; i_alpha input; i_d output; i_beta input; theta_e input
function [i_q,i_d] = park(i_alpha,i_beta,theta_e)

i_d=i_alpha*cos(theta_e)+i_beta*sin(theta_e);
i_q=-i_alpha*sin(theta_e)+i_beta*cos(theta_e);
% I_d=-(I_alph.*cos(theta)+I_beta.*sin(theta));
% I_q= -(-I_alph.*sin(theta)+I_beta.*cos(theta));

== matlab function NGW_model/带摩擦考虑的模型优化/控制系统/反Park变换 ==
  data: u_d input; u_q input; u_alpha output; u_beta output; theta_e input
function [u_alpha, u_beta]  = inv_park(u_d,u_q,theta_e)

u_alpha=cos(theta_e)*u_d-sin(theta_e)*u_q;
u_beta=sin(theta_e)*u_d+cos(theta_e)*u_q;

end
